simulink model "pmdc_hbridge_motor"  (R2024b)
settings: Solver=VariableStepAuto  StartTime=0.0  StopTime=3.0  RelTol=1e-3
PreLoadFcn:
  | init_params;
values from neighbouring files (symbols this model uses):
  A_imb = 0    [generate_dataset.m]    (also in init_params.m)
  Duty = 88    [generate_dataset.m]    (also in init_params.m)
  f_imb = 25    [generate_dataset.m]    (also in init_params.m)
  Kt_motor = 0.055    [generate_dataset.m]    (also in init_params.m)
  R_ext = 1.0    (= 1)    [generate_dataset.m]    (also in init_params.m)
  T0 = 0.05    [generate_dataset.m]    (also in init_params.m)
libraries: fl_lib x9, nesl_utility x6, ee_lib x2
settings Model: Creator=HP  LastModifiedBy=HP

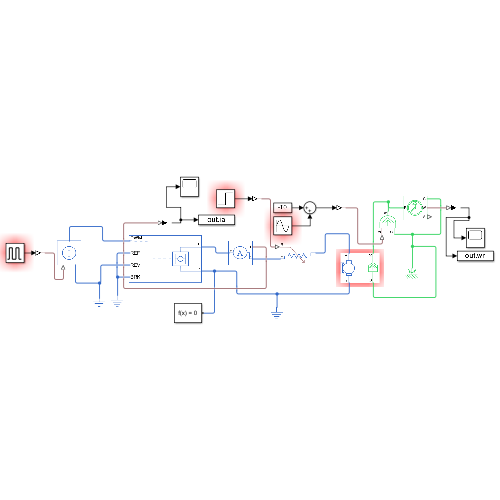
[thumbnail: Simulink's stored preview of the top-level diagram]
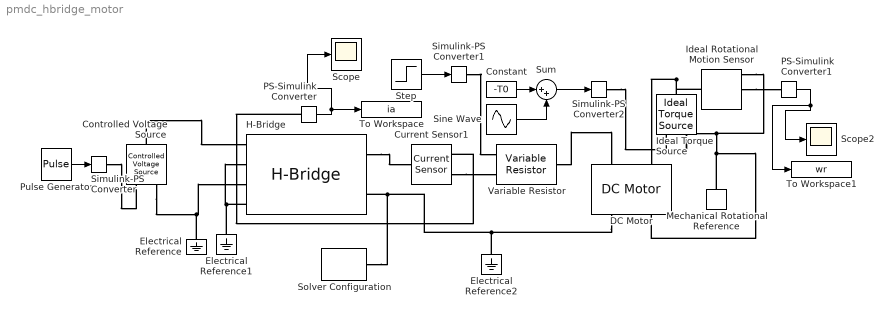
== system pmdc_hbridge_motor ==
  Constant : Constant  Value=-T0
  Controlled Voltage Source : fl_lib/Electrical/Electrical Sources/Controlled Voltage Source
  Current Sensor1 : fl_lib/Electrical/Electrical Sensors/Current Sensor
  DC Motor : ee_lib/Electromechanical/Brushed Motors/DC Motor  field_option=ee.enum.field_option.pm  Rf=100 Ohm  Lf=1 H  Laf=0.15 H  If0=0 A  parameterization=ee.enum.dcparam_option.circuit_param  Ra=1.0 Ohm  La=0.005 H  emf_or_torque=ee.enum.emf_or_torque.ki  Kv=0.055 V*s/rad  Ki=Kt_motor N*m/A  T_stall=0.24e-3 N*m  w_max=19100 rpm  w_rated=15000 rpm  P_rated=0.08 W  V_rated=1.5 V  lam_param=ee.enum.lam_param.damping  i_noload=0 A  V_i_noload=1.5 V  J=2e-4 kg*m^2  lam=1e-5 N*m*s/rad  speed0=0 rpm  t_fault_armature=1 s  t_fault_field=1 s  fault_action=simscape.enum.assert.action.none  alpha=3.93e-3 1/K  Tmeas=25 degC  thermal_mass=100 J/K  initial_temperature=25 degC
  Electrical Reference : fl_lib/Electrical/Electrical Elements/Electrical Reference
  Electrical Reference1 : fl_lib/Electrical/Electrical Elements/Electrical Reference
  Electrical Reference2 : fl_lib/Electrical/Electrical Elements/Electrical Reference
  H-Bridge : ee_lib/Semiconductors & Converters/Converters/H-Bridge  supply_ports=ee.enum.supply_ports.hidesupply  pwm_or_av=ee.enum.pwm_or_av.pwm  regenerative_braking_mode=ee.enum.converters.regenerative_braking_mode.depends_on_rev  discontinuous=ee.enum.current_profile.continuous  freewheeling_mode=ee.enum.converters.freewheeling_mode.one_switch_one_diode  Rload=10 Ohm  Lload=1e-5 H  F=10 kHz  Venable=2.5 V  Vmax=3.3 V  Vreverse=2.5 V  Vbrake=2.5 V  Vm=12 V  Ron=0.1 Ohm  Don=0.05 Ohm  Goff=1e-6 S  Tmeas=298.15 K  Ron2=0.1 Ohm  Don2=0.05 Ohm  Tmeas2=398.15 K  thermal_mass=100 J/K  initial_temperature=298.15 K
  Ideal Rotational Motion Sensor : fl_lib/Mechanical/Mechanical Sensors/Ideal Rotational Motion Sensor  reference=foundation.enum.MeasurementReference.difference  acceleration_port=false  velocity_port=true  position_port=true  wrap_angle=false  offset=0 rad
  Ideal Torque Source : fl_lib/Mechanical/Mechanical Sources/Ideal Torque Source
  Mechanical Rotational Reference : fl_lib/Mechanical/Rotational Elements/Mechanical Rotational Reference
  PS-Simulink Converter : nesl_utility/PS-Simulink Converter  PhysicalDomain=network_engine_domain  SubClassName=ps_output  LeftPortType=input  RightPortType=output  PseudoPeriodic=off  Frequencies=[]  VectorFormat=inherit  Unit=A  AffineConversion=off
  PS-Simulink Converter1 : nesl_utility/PS-Simulink Converter  PhysicalDomain=network_engine_domain  SubClassName=ps_output  LeftPortType=input  RightPortType=output  PseudoPeriodic=off  Frequencies=[]  VectorFormat=inherit  Unit=rad/s  AffineConversion=off
  Pulse Generator : DiscretePulseGenerator  PulseType=Time based  Amplitude=3.3  Period=1e-3  PulseWidth=Duty
  Scope : Scope
  Scope2 : Scope
  Simulink-PS Converter : nesl_utility/Simulink-PS Converter  PhysicalDomain=network_engine_domain  SubClassName=ps_input  LeftPortType=input  RightPortType=output  PseudoPeriodic=off  Frequencies=[]  NoiseDistribution=none  NoiseParameters=[]  Unit=1  AffineConversion=on  FilteringAndDerivatives=provide  SimscapeFilterOrder=1  InputFilterTimeConstant=0.001  UdotUserProvided=0
  Simulink-PS Converter1 : nesl_utility/Simulink-PS Converter  PhysicalDomain=network_engine_domain  SubClassName=ps_input  LeftPortType=input  RightPortType=output  PseudoPeriodic=off  Frequencies=[]  NoiseDistribution=none  NoiseParameters=[]  Unit=Ohm  AffineConversion=off  FilteringAndDerivatives=provide  SimscapeFilterOrder=1  InputFilterTimeConstant=0.001  UdotUserProvided=0
  Simulink-PS Converter2 : nesl_utility/Simulink-PS Converter  PhysicalDomain=network_engine_domain  SubClassName=ps_input  LeftPortType=input  RightPortType=output  PseudoPeriodic=off  Frequencies=[]  NoiseDistribution=none  NoiseParameters=[]  Unit=N*m  AffineConversion=off  FilteringAndDerivatives=provide  SimscapeFilterOrder=1  InputFilterTimeConstant=0.001  UdotUserProvided=0
  Sine Wave : Sin  Amplitude=A_imb  Frequency=2*pi*f_imb  SampleTime=0
  Solver Configuration : nesl_utility/Solver Configuration  PhysicalDomain=network_engine_domain  SubClassName=solver  LeftPortType=input  RightPortType=generic  Tones=[]  Harmonics=[]  SimulateNoise=off  Profile=off  UseLocalSampling=off  EnableSwitchedLinearOptims=on  FrequencyDomain=off  UseCCode=off  RelTol=0.001  AbsTol=0.001  MinStep=1e-09  ToWorkspace=off  RevertToSquareIcSolve=off  NumHomotopyIterations=100  PhasorMode=off  PhasorModeNumHarmonics=1  ConsistencySolver=NEWTON_XTOL_AFTER_FTOL  IndexReductionMethod=DerivativeReplacement  DoDC=off  ResidualTolerance=1e-09  ConsistencyTolSource=GLOBAL  ConsistencyAbsTol=0.001  ConsistencyRelTol=0.001  ConsistencyTolFactor=0.001  UseLocalSolver=off  LocalSolverChoice=NE_BACKWARD_EULER_ADVANCER  ResolveIndetEquations=on  FunctionEvalNumThread=1  LocalSolverSampleTime=0.001  DoFixedCost=off  MaxNonlinIter=3  MaxModeIter=2  ComputeImpulses=off  ImpulseIterations=2  LinearAlgebra=auto  LinearAlgebraNumThread=0  EquationFormulation=NE_TIME_EF  DelaysMemoryBudget=1024  AutomaticFiltering=on  FilteringTimeConstant=0.001  PartitionStorageMethod=AS_NEEDED  PartitionMemoryBudget=1024  PartitionMethod=ROBUST  MultibodyUseLocalSolver=off  MultibodyLocalSolverChoice=ODE1  MultibodyLocalSolverSampleTime=0.001
  Step : Step  Before=R_ext  After=R_ext  SampleTime=0
  Sum : Sum  Inputs=|++
  To Workspace : ToWorkspace  VariableName=ia  SampleTime=1e-4
  To Workspace1 : ToWorkspace  VariableName=wr  SampleTime=1e-4
  Variable Resistor : fl_lib/Electrical/Electrical Elements/Variable Resistor  Rmin=1 Ohm  thermalEnable=false  thermal_mass=1 J/K  i_specify=off  i_priority=None  i=0 A  i_nominal_specify=off  i_nominal_value=1  i_nominal_unit=A  v_specify=off  v_priority=None  v=0 V  v_nominal_specify=off  v_nominal_value=1  v_nominal_unit=V  T_specify=off  T_priority=None  T=300 K  T_nominal_specify=off  T_nominal_value=1  T_nominal_unit=K
  wires:
  Pulse Generator/1 -> Simulink-PS Converter/1
  Step/1 -> Simulink-PS Converter1/1
  PS-Simulink Converter/1 -> Scope/1, To Workspace/1
  Sum/1 -> Simulink-PS Converter2/1
  Constant/1 -> Sum/1
  Sine Wave/1 -> Sum/2
  PS-Simulink Converter1/1 -> To Workspace1/1, Scope2/1
  connections:
  Controlled Voltage Source/LConn1 -- H-Bridge/LConn1
  Controlled Voltage Source/RConn2 -- H-Bridge/LConn3 -- Electrical Reference/LConn1
  H-Bridge/LConn4 -- H-Bridge/LConn2 -- Electrical Reference1/LConn1
  Simulink-PS Converter/RConn1 -- Controlled Voltage Source/RConn1
  H-Bridge/RConn1 -- Current Sensor1/LConn1
  Current Sensor1/RConn2 -- Variable Resistor/LConn2
  Variable Resistor/RConn1 -- DC Motor/LConn1
  Ideal Torque Source/LConn1 -- Ideal Rotational Motion Sensor/LConn1 -- DC Motor/LConn2
  Ideal Torque Source/RConn2 -- Ideal Rotational Motion Sensor/RConn1 -- DC Motor/RConn2 -- Mechanical Rotational Reference/LConn1
  DC Motor/RConn1 -- Electrical Reference2/LConn1 -- Solver Configuration/RConn1 -- H-Bridge/RConn2
  Simulink-PS Converter1/RConn1 -- Variable Resistor/LConn1
  PS-Simulink Converter/LConn1 -- Current Sensor1/RConn1
  Simulink-PS Converter2/RConn1 -- Ideal Torque Source/RConn1
  Ideal Rotational Motion Sensor/RConn2 -- PS-Simulink Converter1/LConn1
